simulink model "mockup"  (R2026b)
settings: Solver=VariableStepAuto  StopTime=inf
undefined symbols (not defined in the file): f
libraries: instrumentlib x1
settings Model: Creator=adiay  LastModifiedBy=adiay

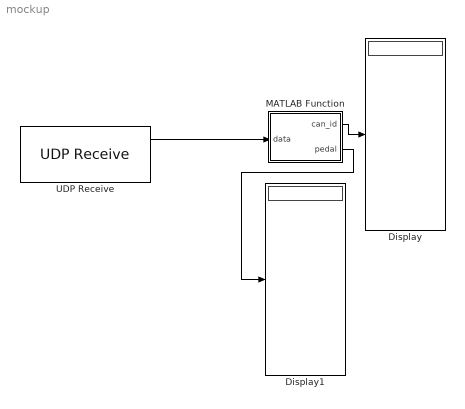
== system mockup ==
  Display : Display
  Display1 : Display
  MATLAB Function : MATLAB Function  TreatAsAtomicUnit=on
  UDP Receive : instrumentlib/UDP Receive  LocalAddress=0.0.0.0  LocalPort=5005  EnablePortSharing=off  Host=0.0.0.0  Port=5006  GetLatestData=off  DataSize=[ 11, 1 ]  DataType=uint8  ASCIIFormatting=%f,  Terminator=LF  CustomTerminator=10  ByteOrder=big-endian  EnableBlockingMode=off  Timeout=10  SampleTime=0.01  SimulateUsing=Interpreted execution
  wires:
  MATLAB Function/1(can_id) -> Display/1
  UDP Receive/1 -> MATLAB Function/1(data)
  MATLAB Function/2(pedal) -> Display1/1

== matlab function mockup/MATLAB Function ==
  data: data input; can_id output; pedal output
function [can_id, pedal] = fcn(data)

can_id = double(data(1)) + 256 * double(data(2));

value = double(data(4)) + 256 * double(data(5));

pedal = value / 10;
